simulink model "ProyectoFinal"  (R2025b)
settings: Solver=VariableStepAuto  StartTime=0.0  StopTime=1e-3  RelTol=1e-3
libraries: fl_lib x20, nesl_utility x6, slpidlib x1
settings Model: Creator=Kevsツ  LastModifiedBy=kevin
settings RTWCC: GPUComputeCapability=3.5

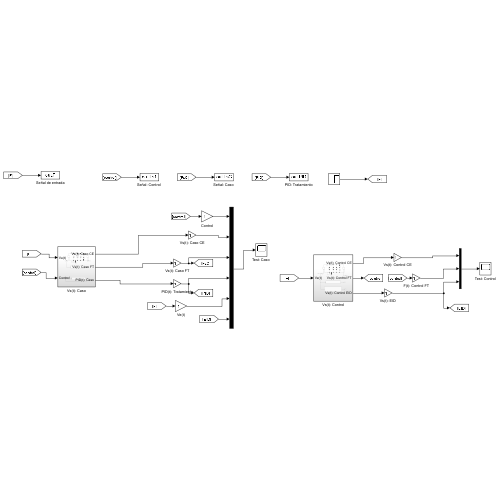
[thumbnail: Simulink's stored preview of the top-level diagram]
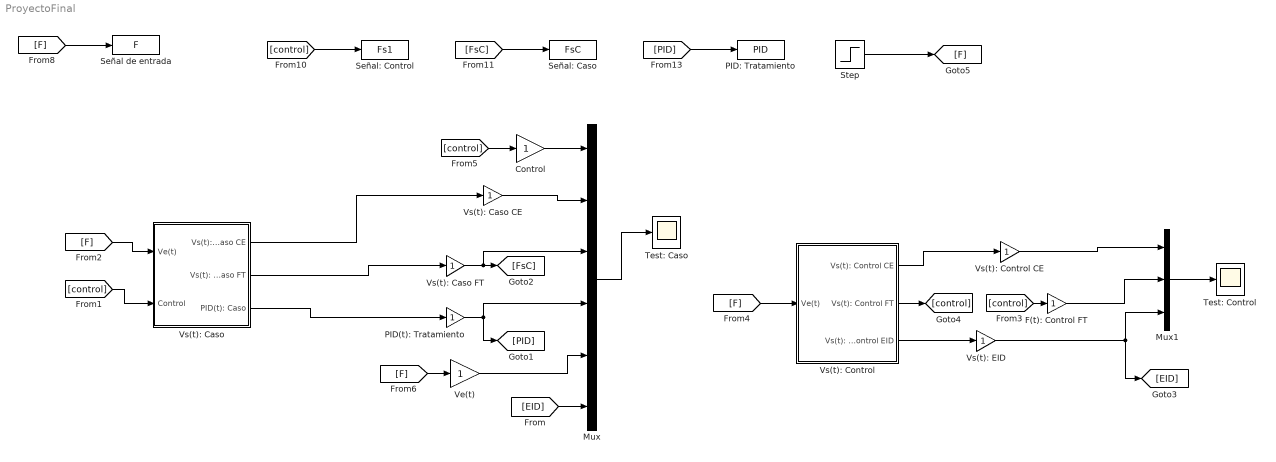
== system ProyectoFinal ==
  Control : Gain
  F(t): Control FT : Gain
  Mux : Mux  Inputs=6
  Mux1 : Mux  Inputs=3
  PID(t): Tratamiento : Gain
  PID: Tratamiento : ToWorkspace  VariableName=PID  SampleTime=-1
  Señal de entrada : ToWorkspace  VariableName=F  SampleTime=-1
  "Señal: Caso " : ToWorkspace  VariableName=FsC  SampleTime=-1
  "Señal: Control " : ToWorkspace  VariableName=Fs1  SampleTime=-1
  Step : Step  Time=1e-4  SampleTime=0
  "Test: Caso " : Scope
      settings: ActiveDisplayYMinimum=-0.12499999999999997  ActiveDisplayYMaximum=1.125
  Test: Control : Scope
      settings: ActiveDisplayYMinimum=-0.125  ActiveDisplayYMaximum=1.125
  Ve(t) : Gain
  Vs(t): Caso : Subsystem
  Vs(t): Caso CE : Gain
  Vs(t): Caso FT : Gain
  Vs(t): Control : Subsystem
  Vs(t): Control CE : Gain
  "Vs(t): EID " : Gain
  wires:
  Mux/1 -> "Test: Caso "/1
  Control/1 -> Mux/1
  Step/1 -> [F]
  Vs(t): Caso/1(Vs(t): Caso CE) -> Vs(t): Caso CE/1
  [F] -> Señal de entrada/1
  [FsC] -> "Señal: Caso "/1
  [control] -> "Señal: Control "/1
  [PID] -> PID: Tratamiento/1
  Vs(t): Caso/2(Vs(t): Caso FT) -> Vs(t): Caso FT/1
  Vs(t): Control/2(Vs(t): Control FT) -> [control]
  [control] -> Vs(t): Caso/2(Control)
  Vs(t): Control/1(Vs(t): Control CE) -> Vs(t): Control CE/1
  Vs(t): Control CE/1 -> Mux1/1
  [control] -> F(t): Control FT/1
  F(t): Control FT/1 -> Mux1/2
  [F] -> Vs(t): Caso/1(Ve(t))
  [F] -> Vs(t): Control/1(Ve(t))
  Mux1/1 -> Test: Control/1
  [control] -> Control/1
  Vs(t): Caso/3(PID(t): Caso) -> PID(t): Tratamiento/1
  Vs(t): Caso CE/1 -> Mux/2
  Vs(t): Caso FT/1 -> Mux/3, [FsC]
  PID(t): Tratamiento/1 -> Mux/4, [PID]
  [F] -> Ve(t)/1
  Ve(t)/1 -> Mux/5
  Vs(t): Control/3(Vs(t): Control EID) -> "Vs(t): EID "/1
  "Vs(t): EID "/1 -> [EID], Mux1/3
  [EID] -> Mux/6

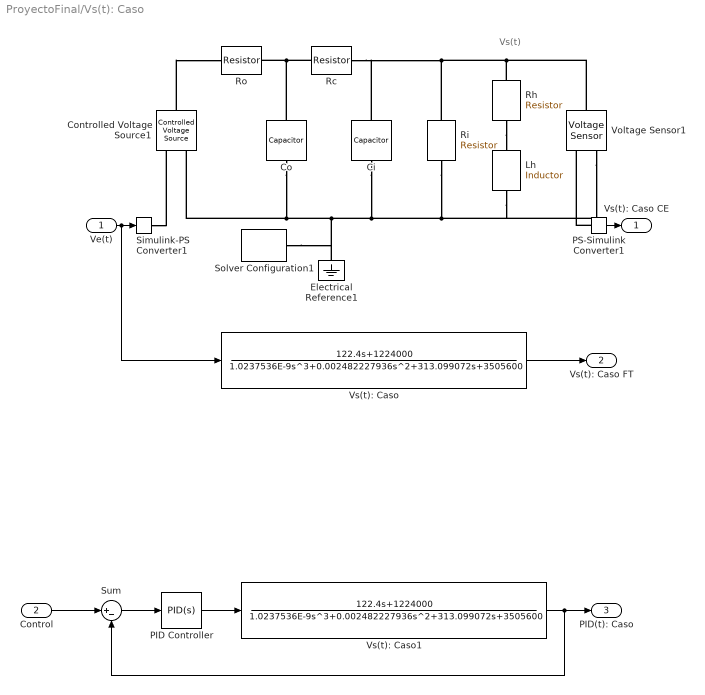
== system ProyectoFinal/Vs(t): Caso ==
  note: Vs(t)
  Ve(t) : Inport
  Control : Inport  Port=2
  Ci : fl_lib/Electrical/Electrical Elements/Capacitor  c=15 nF  r=1e-6 Ohm  g=0 1/Ohm  i_specify=off  i_priority=None  i=0 A  i_nominal_specify=off  i_nominal_value=1  i_nominal_unit=A  v_specify=off  v_priority=None  v=0 V  v_nominal_specify=off  v_nominal_value=1  v_nominal_unit=V  vc_specify=off  vc_priority=High  vc=0 V  vc_nominal_specify=off  vc_nominal_value=1  vc_nominal_unit=V
  Co : fl_lib/Electrical/Electrical Elements/Capacitor  c=6.8 nF  r=1e-6 Ohm  g=0 1/Ohm  i_specify=off  i_priority=None  i=0 A  i_nominal_specify=off  i_nominal_value=1  i_nominal_unit=A  v_specify=off  v_priority=None  v=0 V  v_nominal_specify=off  v_nominal_value=1  v_nominal_unit=V  vc_specify=off  vc_priority=High  vc=0 V  vc_nominal_specify=off  vc_nominal_value=1  vc_nominal_unit=V
  Controlled Voltage Source1 : fl_lib/Electrical/Electrical Sources/Controlled Voltage Source
  Electrical Reference1 : fl_lib/Electrical/Electrical Elements/Electrical Reference
  Lh : fl_lib/Electrical/Electrical Elements/Inductor  l=180 mH  r=0 Ohm  g=1e-9 1/Ohm  i_specify=off  i_priority=None  i=0 A  i_nominal_specify=off  i_nominal_value=1  i_nominal_unit=A  v_specify=off  v_priority=None  v=0 V  v_nominal_specify=off  v_nominal_value=1  v_nominal_unit=V  i_L_specify=off  i_L_priority=High  i_L=0 A  i_L_nominal_specify=off  i_L_nominal_value=1  i_L_nominal_unit=A
  PID Controller : slpidlib/PID Controller  Controller=PID  Form=Parallel  TimeDomain=Continuous-time  UseExternalTs=off  SampleTime=-1  IntegratorMethod=Forward Euler  FilterMethod=Forward Euler  ControllerParametersSource=internal  P=100  I=1E7  UseKiTs=off  D=0  UseExternalDerivativeSource=off  N=100  UseFilter=on  TunerSelectOption=Transfer Function Based (PID Tuner App)  InitialConditionSource=internal  InitialConditionForIntegrator=0  InitialConditionForFilter=0  DifferentiatorICPrevScaledInput=0  ExternalReset=none  TrackingMode=off  Kt=1  LimitOutput=off  SatLimitsSource=internal  UpperSaturationLimit=inf  LowerSaturationLimit=-inf  LinearizeAsGain=on  AntiWindupMode=none  Kb=1  LimitIntegrator=off  UpperIntegratorSaturationLimit=inf  LowerIntegratorSaturationLimit=-inf  POutMin=[]  POutMax=[]  IOutMin=[]  IOutMax=[]  DOutMin=[]  DOutMax=[]  NOutMin=[]  NOutMax=[]  SumOutMin=[]  SumOutMax=[]  SaturationOutMin=[]  SaturationOutMax=[]  PParamMin=[]  PParamMax=[]  IParamMin=[]  IParamMax=[]  DParamMin=[]  DParamMax=[]  NParamMin=[]  NParamMax=[]  KbParamMin=[]  KbParamMax=[]  KtParamMin=[]  KtParamMax=[]  KbOutMin=[]  KbOutMax=[]  KtOutMin=[]  KtOutMax=[]  IntegratorOutMin=[]  IntegratorOutMax=[]  FilterOutMin=[]  FilterOutMax=[]  SumI1OutMin=[]  SumI1OutMax=[]  SumI2OutMin=[]  SumI2OutMax=[]  SumI3OutMin=[]  SumI3OutMax=[]  SumI4OutMin=[]  SumI4OutMax=[]  SumDOutMin=[]  SumDOutMax=[]  DifferentiatorOutMin=[]  DifferentiatorOutMax=[]  FilterDiffOutCoefMin=[]  FilterDiffOutCoefMax=[]  ReciprocalOutMin=[]  ReciprocalOutMax=[]  SumDenOutMin=[]  SumDenOutMax=[]  SumNumOutMin=[]  SumNumOutMax=[]  DivideOutMin=[]  DivideOutMax=[]  UdiffTsProdOutMin=[]  UdiffTsProdOutMax=[]  NTsProdOutMin=[]  NTsProdOutMax=[]  UintegralTsProdOutMin=[]  UintegralTsProdOutMax=[]  UngainTsProdOutMin=[]  UngainTsProdOutMax=[]  ClampingZeroOutDataTypeStr=Inherit: Inherit via back propagation  ClampingZeroOutMin=[]  ClampingZeroOutMax=[]  FilterDenConstantOutDataTypeStr=Inherit: Inherit via back propagation  FilterDenConstantOutMin=[]  FilterDenConstantOutMax=[]  PCopyOutDataTypeStr=Inherit: Inherit via back propagation  PCopyOutMin=[]  PCopyOutMax=[]  NCopyOutDataTypeStr=Inherit: Inherit via back propagation  NCopyOutMin=[]  NCopyOutMax=[]  IntegratorContinuousStateAttributes=''  IntegratorStateMustResolveToSignalObject=off  IntegratorRTWStateStorageClass=Auto  FilterContinuousStateAttributes=''  FilterStateMustResolveToSignalObject=off  FilterRTWStateStorageClass=Auto  ParallelPVariant=InternalParameters  IdealPVariant=Disabled  IVariant=InternalParameters  DVariant=InternalParameters  IntegratorVariant=Continuous  SatVariant=Disabled  AWVariant=Passthrough  PCopyVariant=Disabled  TRVariant=Disabled  FdbkBlocksVariant=Forward  IdealPFdbkVariant=Disabled  SatFdbkVariant=Disabled  DerivativeFilterVariant=ContFilter  NVariant=InternalParameters  NCopyVariant=Disabled  FilterICVariant=InternalICsFilter  IntegratorICVariant=InternalICs  ExternalResetVariant=Disabled  TRSumVariant=Passthrough  SumFdbkVariant=Disabled  SumVariant=Sum_PID  TsampFilterVariant=InternalTs  TsampNgainVariant=Passthrough  TsampIntegralVariant=Disabled_SignalSpec  ExternalSaturationOutDataTypeStr=Inherit: Same as second input  DerivativeSourceVariant=ErrorSignal  PreIntVariant=InternalPreInt
  PS-Simulink Converter1 : nesl_utility/PS-Simulink Converter  PhysicalDomain=network_engine_domain  SubClassName=ps_output  LeftPortType=input  RightPortType=output  PseudoPeriodic=off  Frequencies=[]  VectorFormat=inherit  Unit=inherit  AffineConversion=off
  Rc : fl_lib/Electrical/Electrical Elements/Resistor  R=100 Ohm  i_specify=off  i_priority=None  i=0 A  i_nominal_specify=off  i_nominal_value=1  i_nominal_unit=A  v_specify=off  v_priority=None  v=0 V  v_nominal_specify=off  v_nominal_value=1  v_nominal_unit=V
  Rh : fl_lib/Electrical/Electrical Elements/Resistor  R=1.8 kOhm  i_specify=off  i_priority=None  i=0 A  i_nominal_specify=off  i_nominal_value=1  i_nominal_unit=A  v_specify=off  v_priority=None  v=0 V  v_nominal_specify=off  v_nominal_value=1  v_nominal_unit=V
  Ri : fl_lib/Electrical/Electrical Elements/Resistor  R=680 Ohm  i_specify=off  i_priority=None  i=0 A  i_nominal_specify=off  i_nominal_value=1  i_nominal_unit=A  v_specify=off  v_priority=None  v=0 V  v_nominal_specify=off  v_nominal_value=1  v_nominal_unit=V
  Ro : fl_lib/Electrical/Electrical Elements/Resistor  R=820 Ohm  i_specify=off  i_priority=None  i=0 A  i_nominal_specify=off  i_nominal_value=1  i_nominal_unit=A  v_specify=off  v_priority=None  v=0 V  v_nominal_specify=off  v_nominal_value=1  v_nominal_unit=V
  Simulink-PS Converter1 : nesl_utility/Simulink-PS Converter  PhysicalDomain=network_engine_domain  SubClassName=ps_input  LeftPortType=input  RightPortType=output  PseudoPeriodic=off  Frequencies=[]  NoiseDistribution=none  NoiseParameters=[]  Unit=1  AffineConversion=off  FilteringAndDerivatives=provide  SimscapeFilterOrder=1  InputFilterTimeConstant=0.001  UdotUserProvided=0
  Solver Configuration1 : nesl_utility/Solver Configuration  PhysicalDomain=network_engine_domain  SubClassName=solver  LeftPortType=input  RightPortType=generic  Tones=[]  Harmonics=[]  SimulateNoise=off  Profile=off  UseLocalSampling=off  EnableSwitchedLinearOptims=on  FrequencyDomain=off  UseCCode=off  RelTol=0.001  AbsTol=0.001  MinStep=1e-09  ToWorkspace=off  RevertToSquareIcSolve=off  NumHomotopyIterations=100  PhasorMode=off  PhasorModeNumHarmonics=1  ConsistencySolver=NEWTON_XTOL_AFTER_FTOL  IndexReductionMethod=DerivativeReplacement  DoDC=off  ResidualTolerance=1e-09  ConsistencyTolSource=GLOBAL  ConsistencyAbsTol=0.001  ConsistencyRelTol=0.001  ConsistencyTolFactor=0.001  UseLocalSolver=off  LocalSolverChoice=NE_BACKWARD_EULER_ADVANCER  ResolveIndetEquations=on  FunctionEvalNumThread=1  LocalSolverSampleTime=0.001  DoFixedCost=off  MaxNonlinIter=3  MaxModeIter=2  ComputeImpulses=off  ImpulseIterations=2  LinearAlgebra=auto  LinearAlgebraNumThread=0  EquationFormulation=NE_TIME_EF  DelaysMemoryBudget=1024  AutomaticFiltering=on  FilteringTimeConstant=0.001  PartitionStorageMethod=AS_NEEDED  PartitionMemoryBudget=1024  PartitionMethod=ROBUST  MultibodyUseLocalSolver=off  MultibodyLocalSolverChoice=ODE1  MultibodyLocalSolverSampleTime=0.001
  Sum : Sum  Inputs=|+-
  Voltage Sensor1 : fl_lib/Electrical/Electrical Sensors/Voltage Sensor
  Vs(t): Caso : TransferFcn  Numerator=[122.4, 1224000]  Denominator=[1.0237536E-9, 0.002482227936, 313.099072, 3505600]
  Vs(t): Caso1 : TransferFcn  Numerator=[122.4, 1224000]  Denominator=[1.0237536E-9, 0.002482227936, 313.099072, 3505600]
  Vs(t): Caso CE : Outport
  Vs(t): Caso FT : Outport  Port=2
  PID(t): Caso : Outport  Port=3
  wires:
  PS-Simulink Converter1/1 -> Vs(t): Caso CE/1
  Ve(t)/1 -> Vs(t): Caso/1, Simulink-PS Converter1/1
  Vs(t): Caso/1 -> Vs(t): Caso FT/1
  Vs(t): Caso1/1 -> PID(t): Caso/1, Sum/2
  PID Controller/1 -> Vs(t): Caso1/1
  Sum/1 -> PID Controller/1
  Control/1 -> Sum/1
  connections:
  Voltage Sensor1/LConn1 -- Rh/LConn1 -- Rc/RConn1 -- Ci/LConn1 -- Ri/LConn1
  Ci/RConn1 -- Lh/RConn1 -- Voltage Sensor1/RConn2 -- Ri/RConn1 -- Electrical Reference1/LConn1 -- Solver Configuration1/RConn1 -- Co/RConn1 -- Controlled Voltage Source1/RConn2
  Co/LConn1 -- Rc/LConn1 -- Ro/RConn1
  Controlled Voltage Source1/LConn1 -- Ro/LConn1
  PS-Simulink Converter1/LConn1 -- Voltage Sensor1/RConn1
  Simulink-PS Converter1/RConn1 -- Controlled Voltage Source1/RConn1
  Rh/RConn1 -- Lh/LConn1

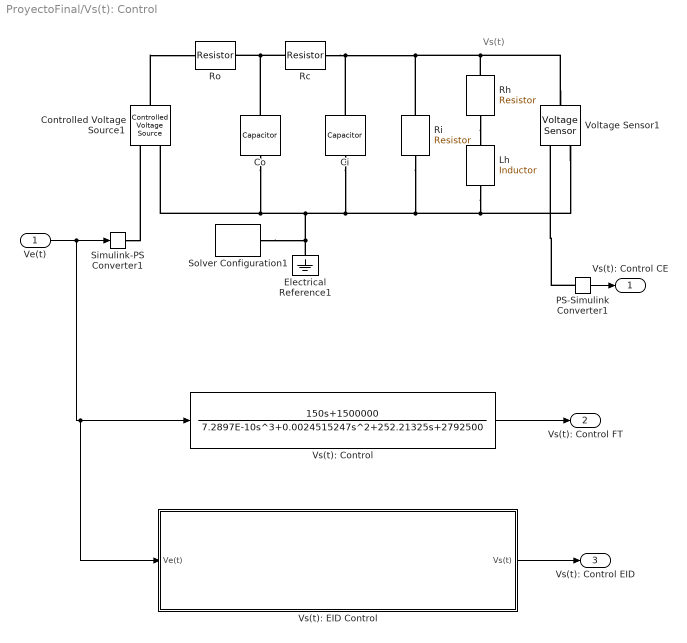
== system ProyectoFinal/Vs(t): Control ==
  note: Vs(t)
  Ve(t) : Inport
  Ci : fl_lib/Electrical/Electrical Elements/Capacitor  c=22 nF  r=1e-6 Ohm  g=0 1/Ohm  i_specify=off  i_priority=None  i=0 A  i_nominal_specify=off  i_nominal_value=1  i_nominal_unit=A  v_specify=off  v_priority=None  v=0 V  v_nominal_specify=off  v_nominal_value=1  v_nominal_unit=V  vc_specify=off  vc_priority=High  vc=0 V  vc_nominal_specify=off  vc_nominal_value=1  vc_nominal_unit=V
  Co : fl_lib/Electrical/Electrical Elements/Capacitor  c=10 nF  r=1e-6 Ohm  g=0 1/Ohm  i_specify=off  i_priority=None  i=0 A  i_nominal_specify=off  i_nominal_value=1  i_nominal_unit=A  v_specify=off  v_priority=None  v=0 V  v_nominal_specify=off  v_nominal_value=1  v_nominal_unit=V  vc_specify=off  vc_priority=High  vc=0 V  vc_nominal_specify=off  vc_nominal_value=1  vc_nominal_unit=V
  Controlled Voltage Source1 : fl_lib/Electrical/Electrical Sources/Controlled Voltage Source
  Electrical Reference1 : fl_lib/Electrical/Electrical Elements/Electrical Reference
  Lh : fl_lib/Electrical/Electrical Elements/Inductor  l=150 mH  r=0 Ohm  g=1e-9 1/Ohm  i_specify=off  i_priority=None  i=0 A  i_nominal_specify=off  i_nominal_value=1  i_nominal_unit=A  v_specify=off  v_priority=None  v=0 V  v_nominal_specify=off  v_nominal_value=1  v_nominal_unit=V  i_L_specify=off  i_L_priority=High  i_L=0 A  i_L_nominal_specify=off  i_L_nominal_value=1  i_L_nominal_unit=A
  PS-Simulink Converter1 : nesl_utility/PS-Simulink Converter  PhysicalDomain=network_engine_domain  SubClassName=ps_output  LeftPortType=input  RightPortType=output  PseudoPeriodic=off  Frequencies=[]  VectorFormat=inherit  Unit=inherit  AffineConversion=off
  Rc : fl_lib/Electrical/Electrical Elements/Resistor  R=47 Ohm  i_specify=off  i_priority=None  i=0 A  i_nominal_specify=off  i_nominal_value=1  i_nominal_unit=A  v_specify=off  v_priority=None  v=0 V  v_nominal_specify=off  v_nominal_value=1  v_nominal_unit=V
  Rh : fl_lib/Electrical/Electrical Elements/Resistor  R=1.5 kOhm  i_specify=off  i_priority=None  i=0 A  i_nominal_specify=off  i_nominal_value=1  i_nominal_unit=A  v_specify=off  v_priority=None  v=0 V  v_nominal_specify=off  v_nominal_value=1  v_nominal_unit=V
  Ri : fl_lib/Electrical/Electrical Elements/Resistor  R=1 kOhm  i_specify=off  i_priority=None  i=0 A  i_nominal_specify=off  i_nominal_value=1  i_nominal_unit=A  v_specify=off  v_priority=None  v=0 V  v_nominal_specify=off  v_nominal_value=1  v_nominal_unit=V
  Ro : fl_lib/Electrical/Electrical Elements/Resistor  R=470 Ohm  i_specify=off  i_priority=None  i=0 A  i_nominal_specify=off  i_nominal_value=1  i_nominal_unit=A  v_specify=off  v_priority=None  v=0 V  v_nominal_specify=off  v_nominal_value=1  v_nominal_unit=V
  Simulink-PS Converter1 : nesl_utility/Simulink-PS Converter  PhysicalDomain=network_engine_domain  SubClassName=ps_input  LeftPortType=input  RightPortType=output  PseudoPeriodic=off  Frequencies=[]  NoiseDistribution=none  NoiseParameters=[]  Unit=1  AffineConversion=off  FilteringAndDerivatives=provide  SimscapeFilterOrder=1  InputFilterTimeConstant=0.001  UdotUserProvided=0
  Solver Configuration1 : nesl_utility/Solver Configuration  PhysicalDomain=network_engine_domain  SubClassName=solver  LeftPortType=input  RightPortType=generic  Tones=[]  Harmonics=[]  SimulateNoise=off  Profile=off  UseLocalSampling=off  EnableSwitchedLinearOptims=on  FrequencyDomain=off  UseCCode=off  RelTol=0.001  AbsTol=0.001  MinStep=1e-09  ToWorkspace=off  RevertToSquareIcSolve=off  NumHomotopyIterations=100  PhasorMode=off  PhasorModeNumHarmonics=1  ConsistencySolver=NEWTON_XTOL_AFTER_FTOL  IndexReductionMethod=DerivativeReplacement  DoDC=off  ResidualTolerance=1e-09  ConsistencyTolSource=GLOBAL  ConsistencyAbsTol=0.001  ConsistencyRelTol=0.001  ConsistencyTolFactor=0.001  UseLocalSolver=off  LocalSolverChoice=NE_BACKWARD_EULER_ADVANCER  ResolveIndetEquations=on  FunctionEvalNumThread=1  LocalSolverSampleTime=0.001  DoFixedCost=off  MaxNonlinIter=3  MaxModeIter=2  ComputeImpulses=off  ImpulseIterations=2  LinearAlgebra=auto  LinearAlgebraNumThread=0  EquationFormulation=NE_TIME_EF  DelaysMemoryBudget=1024  AutomaticFiltering=on  FilteringTimeConstant=0.001  PartitionStorageMethod=AS_NEEDED  PartitionMemoryBudget=1024  PartitionMethod=ROBUST  MultibodyUseLocalSolver=off  MultibodyLocalSolverChoice=ODE1  MultibodyLocalSolverSampleTime=0.001
  Voltage Sensor1 : fl_lib/Electrical/Electrical Sensors/Voltage Sensor
  Vs(t): Control : TransferFcn  Numerator=[150, 1500000]  Denominator=[7.2897E-10, 0.0024515247, 252.21325, 2792500]
  Vs(t): EID Control : Subsystem
  Vs(t): Control CE : Outport
  Vs(t): Control FT : Outport  Port=2
  Vs(t): Control EID : Outport  Port=3
  wires:
  PS-Simulink Converter1/1 -> Vs(t): Control CE/1
  Vs(t): Control/1 -> Vs(t): Control FT/1
  Vs(t): EID Control/1(Vs(t)) -> Vs(t): Control EID/1
  Ve(t)/1 -> Vs(t): EID Control/1(Ve(t)), Vs(t): Control/1, Simulink-PS Converter1/1
  connections:
  Electrical Reference1/LConn1 -- Solver Configuration1/RConn1 -- Lh/RConn1 -- Voltage Sensor1/RConn2 -- Ri/RConn1 -- Ci/RConn1 -- Co/RConn1 -- Controlled Voltage Source1/RConn2
  PS-Simulink Converter1/LConn1 -- Voltage Sensor1/RConn1
  Controlled Voltage Source1/LConn1 -- Ro/LConn1
  Simulink-PS Converter1/RConn1 -- Controlled Voltage Source1/RConn1
  Co/LConn1 -- Rc/LConn1 -- Ro/RConn1
  Ri/LConn1 -- Rh/LConn1 -- Voltage Sensor1/LConn1 -- Rc/RConn1 -- Ci/LConn1
  Rh/RConn1 -- Lh/LConn1

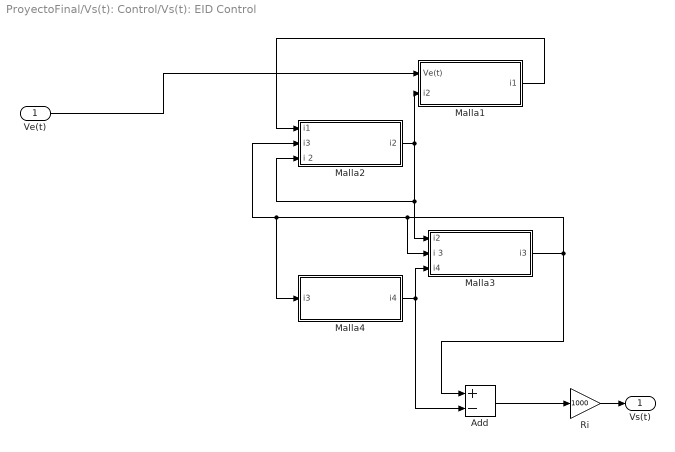
== system ProyectoFinal/Vs(t): Control/Vs(t): EID Control ==
  Ve(t) : Inport
  Add : Sum  Inputs=+-
  Malla1 : Subsystem
  Malla2 : Subsystem
  Malla3 : Subsystem
  Malla4 : Subsystem
  Ri : Gain  Gain=1000
  Vs(t) : Outport
  wires:
  Malla2/1(i2) -> Malla1/2(i2), Malla3/1(i2), Malla2/3(i 2)
  Ve(t)/1 -> Malla1/1(Ve(t))
  Malla1/1(i1) -> Malla2/1(i1)
  Malla3/1(i3) -> Malla4/1(i3), Malla2/2(i3), Malla3/2(i 3), Add/1
  Malla4/1(i4) -> Malla3/3(i4), Add/2
  Ri/1 -> Vs(t)/1
  Add/1 -> Ri/1

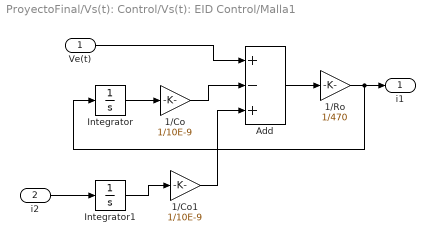
== system ProyectoFinal/Vs(t): Control/Vs(t): EID Control/Malla1 ==
  Ve(t) : Inport
  i2 : Inport  Port=2
  1/Co : Gain  Gain=1/10E-9
  1/Co1 : Gain  Gain=1/10E-9
  1/Ro : Gain  Gain=1/470
  Add : Sum  Inputs=+-+
  Integrator : Integrator
  Integrator1 : Integrator
  i1 : Outport
  wires:
  Ve(t)/1 -> Add/1
  1/Co/1 -> Add/2
  1/Co1/1 -> Add/3
  Integrator1/1 -> 1/Co1/1
  Add/1 -> 1/Ro/1
  i2/1 -> Integrator1/1
  1/Ro/1 -> Integrator/1, i1/1
  Integrator/1 -> 1/Co/1

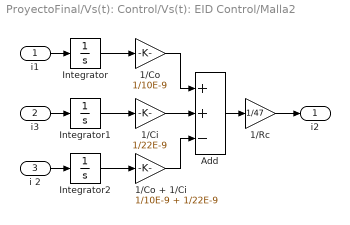
== system ProyectoFinal/Vs(t): Control/Vs(t): EID Control/Malla2 ==
  i1 : Inport
  i3 : Inport  Port=2
  i 2 : Inport  Port=3
  1/Ci : Gain  Gain=1/22E-9
  1/Co : Gain  Gain=1/10E-9
  1/Co + 1/Ci : Gain  Gain=1/10E-9 + 1/22E-9
  1/Rc : Gain  Gain=1/47
  Add : Sum  Inputs=++-
  Integrator : Integrator
  Integrator1 : Integrator
  Integrator2 : Integrator
  i2 : Outport
  wires:
  i1/1 -> Integrator/1
  i3/1 -> Integrator1/1
  1/Co + 1/Ci/1 -> Add/3
  Integrator2/1 -> 1/Co + 1/Ci/1
  Integrator1/1 -> 1/Ci/1
  1/Ci/1 -> Add/2
  Integrator/1 -> 1/Co/1
  1/Co/1 -> Add/1
  i 2/1 -> Integrator2/1
  Add/1 -> 1/Rc/1
  1/Rc/1 -> i2/1

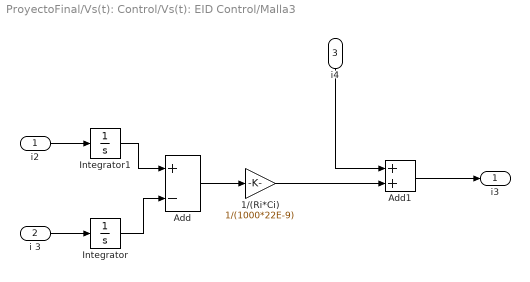
== system ProyectoFinal/Vs(t): Control/Vs(t): EID Control/Malla3 ==
  i2 : Inport
  i 3 : Inport  Port=2
  i4 : Inport  Port=3
  1/(Ri*Ci) : Gain  Gain=1/(1000*22E-9)
  Add : Sum  Inputs=+-
  Add1 : Sum
  Integrator : Integrator
  Integrator1 : Integrator
  i3 : Outport
  wires:
  i2/1 -> Integrator1/1
  Integrator1/1 -> Add/1
  Integrator/1 -> Add/2
  Add/1 -> 1/(Ri*Ci)/1
  1/(Ri*Ci)/1 -> Add1/2
  i4/1 -> Add1/1
  Add1/1 -> i3/1
  i 3/1 -> Integrator/1

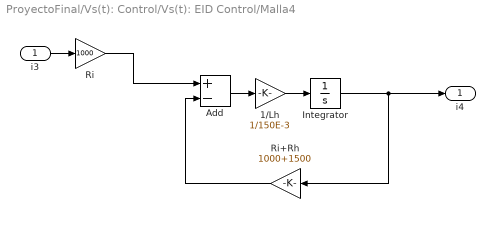
== system ProyectoFinal/Vs(t): Control/Vs(t): EID Control/Malla4 ==
  i3 : Inport
  1/Lh : Gain  Gain=1/150E-3
  Add : Sum  Inputs=+-
  Integrator : Integrator
  Ri : Gain  Gain=1000
  Ri+Rh : Gain  Gain=1000+1500
  i4 : Outport
  wires:
  i3/1 -> Ri/1
  Ri/1 -> Add/1
  Add/1 -> 1/Lh/1
  1/Lh/1 -> Integrator/1
  Ri+Rh/1 -> Add/2
  Integrator/1 -> Ri+Rh/1, i4/1
